simulink model "CLLC"  (R2024a)
settings: Solver=FixedStepAuto  StartTime=0.0  StopTime=0.02  FixedStep=50e-9  RelTol=1e-3
undefined symbols (not defined in the file): DiscIntNeverNeededParam, Ion, Lithium
libraries: spsMosfetLib x8, spsSeriesRLCBranchLib x3, slpidlib x2, simulink x2, spsCurrentMeasurementLib x2, spsBatteryLib x1, spsDCVoltageSourceLib x1, spsLinearTransformerLib x1, spsVoltageMeasurementLib x1, sps_lib x1
settings Model: Creator=DIPAK PRODHANI  LastModifiedBy=DIPAK PRODHANI

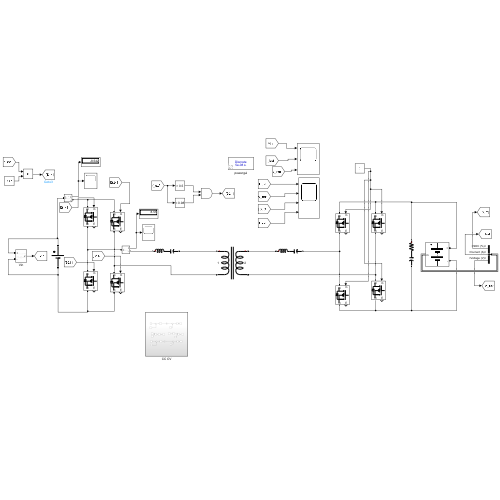
[thumbnail: Simulink's stored preview of the top-level diagram]
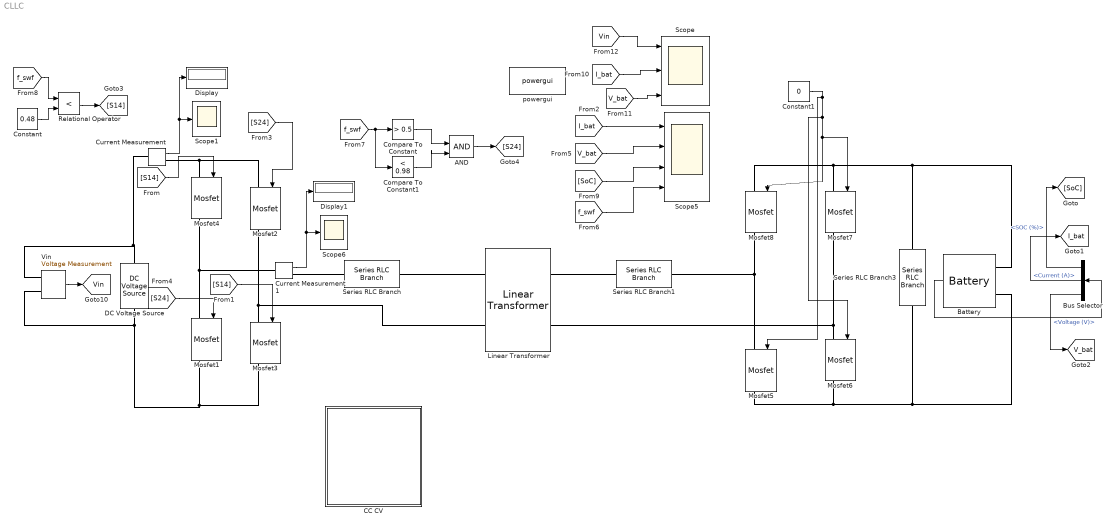
== system CLLC ==
  AND : Logic  IconShape=distinctive  AllPortsSameDT=off  OutDataTypeStr=boolean
  Battery : spsBatteryLib/Battery  BatType=Lithium-Ion  ShowTempParam=off  ThermalPreset=no  ShowAgeParam=off  NomV=720  NomQ=0.0002  SOC=90  Batt_Tr=1e-4  PresetModel=off  MaxQ=0.0002  MinV=540  FullV=838.0707  Dis_rate=8.6957e-05  R=0.5  Normal_OP=0.00018087  expZone="[777.8778  9.826087e-06]"  current=[6.5 13 32.5]  Units=Time  Tci=20  NomT=20  T2=-30  MaxQ2=4.8  FullV2=7.1  Normal_OP2=5.655  expZone2="[6.58           1]"  Rca=0.6  ti=2000  Dp=0  Neq0=0  Tsim=1e6  Ta1=25  Qeol=5.4*0.9  Reol=0.013333*1.2  Char_age=[2.3478, 3]  Dis_age=[2.3478, 10]  N1=1500  N2=10500  N3=1000  N4=1400  Ta2=45  N5=950
  Bus Selector : BusSelector  OutputSignals=SOC (%),Current (A),Voltage (V)
  CC CV : Subsystem
  Compare To Constant : simulink/Logic and Bit Operations/Compare To Constant  relop=>  const=0.5  OutDataTypeStr=boolean
  Compare To Constant1 : simulink/Logic and Bit Operations/Compare To Constant  relop=<  const=0.98  OutDataTypeStr=boolean
  Constant : Constant  Value=0.48
  Constant1 : Constant  Value=0
  Current Measurement : spsCurrentMeasurementLib/Current Measurement  PhasorSimulation=off  OutputType=Complex  PSBequivalent=0
  Current Measurement1 : spsCurrentMeasurementLib/Current Measurement  PhasorSimulation=off  OutputType=Complex  PSBequivalent=0
  DC Voltage Source : spsDCVoltageSourceLib/DC Voltage Source  Amplitude=400  Measurements=None
  Display : Display
  Display1 : Display
  Linear Transformer : spsLinearTransformerLib/Linear Transformer  UNITS=SI  NominalPower=[ 2000 100e3 ]  winding1=[400 0.05 0]  winding2=[615.38 0.1 0]  ThreeWindings=off  winding3=[3.15e+05 0.7938 0.084225]  RmLm=[5000 105.6e-6]  Measurements=None  DataType=on
  Mosfet{1..4} (4 alike) : spsMosfetLib/Mosfet  Ron=0.065  Lon=0  Rd=0.05  Vfd=0.7  IC=0  Rs=1e5  Cs=inf  Measurements=on
  Mosfet{5..8} (4 alike) : spsMosfetLib/Mosfet  Ron=0.08  Lon=0  Rd=0.01  Vfd=0.7  IC=0  Rs=1e5  Cs=inf  Measurements=on
  Relational Operator : RelationalOperator  Operator=<  OutDataTypeStr=boolean  RndMeth=Simplest  InputSameDT=off
  Scope : Scope  NumInputPorts=3
  Scope1 : Scope
  Scope5 : Scope  NumInputPorts=4
  Scope6 : Scope
  Series RLC Branch : spsSeriesRLCBranchLib/Series RLC Branch  LConnTagsString=__new0  RConnTagsString=__new0  BranchType=LC  Resistance=1  Inductance=35.2e-6  SetiL0=off  InitialCurrent=0  Capacitance=71e-9  Setx0=off  InitialVoltage=0  Measurements=None
  Series RLC Branch1 : spsSeriesRLCBranchLib/Series RLC Branch  LConnTagsString=__new0  RConnTagsString=__new0  BranchType=LC  Resistance=1  Inductance=83.31e-6  SetiL0=off  InitialCurrent=0  Capacitance=30e-6  Setx0=off  InitialVoltage=0  Measurements=None
  Series RLC Branch3 : spsSeriesRLCBranchLib/Series RLC Branch  LConnTagsString=__new0  RConnTagsString=__new0  BranchType=RC  Resistance=0.02  Inductance=1e-3  SetiL0=off  InitialCurrent=0  Capacitance=100e-6  Setx0=off  InitialVoltage=0  Measurements=None
  Vin : spsVoltageMeasurementLib/Voltage Measurement  PhasorSimulation=off  OutputType=Complex  PSBequivalent=0
  powergui : sps_lib/powergui  Priority=1  SimulationMode=Discrete  SampleTime=50e-9  frequency=60  Iterations=50  frequencyindice=0  Pbase=100e6  ErrMax=1e-4  UnitsV=kV  UnitsW=MW  buscounter=0  FunctionMessages=off  echomessages=off  EnableUseOfTLC=off  CurrentSourceSwitches=off  DisableSnubberDevices=off  DisableRonSwitches=off  DisableVfSwitches=off  DisplayEquations=off  AutomaticDiscreteSolvers=off  SolverType=Tustin/Backward Euler (TBE)  Interpol=off  ExternalGateDelay=off  methode=off  Ts=100  x0status=blocks  SPID=on  SwTol=0  HookPort=off  NonlinearTolerance=1e-4  nMaxIteration=100  ContinueOnMaxIteration=off  RestoreLinks=warning  ResistiveCurrentMeasurement=off  Frange=[0:2:500]  Ylog=off  Xlog=on  ShowGrid=off  save=off  variable=ZData  structure=0  ZoomFFT=off  StartTime=0.0  cycles=1  DisplayStyle=1  fundamental=60  FreqAxis=off  MaxFrequency=1000  frequencyindicesteady=1  RmsSteady=1  display=off
  tag scope: I_bat=global, V_bat=global, Vin=global
  wires:
  Vin/1 -> [Vin]
  Battery/1 -> Bus Selector/1
  Current Measurement/1 -> Display/1, Scope1/1
  Current Measurement1/1 -> Display1/1, Scope6/1
  Bus Selector/1 -> [SoC]  "<SOC (%)>"
  Bus Selector/2 -> [I_bat]  "<Current (A)>"
  Bus Selector/3 -> [V_bat]  "<Voltage (V)>"
  [f_swf] -> Relational Operator/1
  Constant/1 -> Relational Operator/2
  Relational Operator/1 -> [S14]
  [S14] -> Mosfet4/1
  [S14] -> Mosfet3/1
  [f_swf] -> Compare To Constant1/1, Compare To Constant/1
  Compare To Constant/1 -> AND/1
  Compare To Constant1/1 -> AND/2
  AND/1 -> [S24]
  [S24] -> Mosfet2/1
  [S24] -> Mosfet1/1
  [V_bat] -> Scope/3
  [I_bat] -> Scope/2
  Constant1/1 -> Mosfet5/1, Mosfet6/1, Mosfet7/1, Mosfet8/1
  [I_bat] -> Scope5/1
  [V_bat] -> Scope5/2
  [f_swf] -> Scope5/4
  [SoC] -> Scope5/3
  [Vin] -> Scope/1
  connections:
  Series RLC Branch3/LConn1 -- Battery/LConn1 -- Mosfet7/LConn1 -- Mosfet8/LConn1
  Series RLC Branch3/RConn1 -- Battery/LConn2 -- Mosfet5/RConn1 -- Mosfet6/RConn1
  DC Voltage Source/LConn1 -- Mosfet3/RConn1 -- Mosfet1/RConn1 -- Vin/LConn2
  Linear Transformer/LConn2 -- Mosfet2/RConn1 -- Mosfet3/LConn1
  Linear Transformer/RConn2 -- Mosfet6/LConn1 -- Mosfet7/RConn1
  Vin/LConn1 -- Current Measurement/LConn1 -- DC Voltage Source/RConn1
  Mosfet8/RConn1 -- Series RLC Branch1/RConn1 -- Mosfet5/LConn1
  Mosfet1/LConn1 -- Current Measurement1/LConn1 -- Mosfet4/RConn1
  Series RLC Branch/RConn1 -- Linear Transformer/LConn1
  Series RLC Branch1/LConn1 -- Linear Transformer/RConn1
  Mosfet2/LConn1 -- Current Measurement/RConn1 -- Mosfet4/LConn1
  Current Measurement1/RConn1 -- Series RLC Branch/LConn1

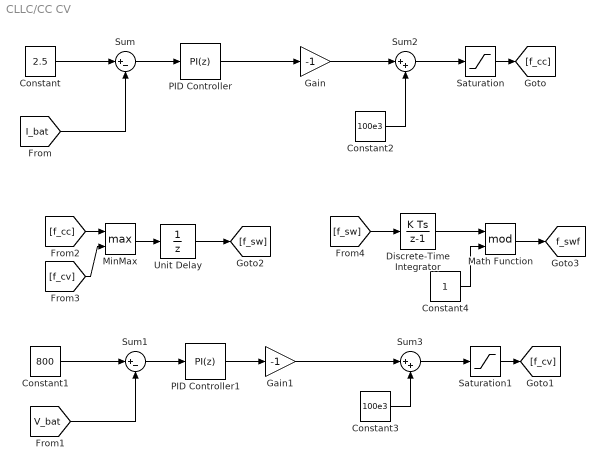
== system CLLC/CC CV ==
  Constant : Constant  Value=2.5
  Constant1 : Constant  Value=800
  Constant2 : Constant  Value=100e3
  Constant3 : Constant  Value=100e3
  Constant4 : Constant
  Discrete-Time Integrator : DiscreteIntegrator  SampleTime=50e-9  ICPrevOutput=DiscIntNeverNeededParam  ICPrevScaledInput=DiscIntNeverNeededParam
  Gain : Gain  Gain=-1
  Gain1 : Gain  Gain=-1
  Math Function : Math  Operator=mod
  MinMax : MinMax  Function=max  Inputs=2
  PID Controller : slpidlib/PID Controller  Controller=PI  Form=Parallel  TimeDomain=Discrete-time  UseExternalTs=off  SampleTime=50e-9  IntegratorMethod=Forward Euler  FilterMethod=Forward Euler  ControllerParametersSource=internal  P=2000  I=500000  UseKiTs=off  D=0  UseExternalDerivativeSource=off  N=100  UseFilter=on  TunerSelectOption=Transfer Function Based (PID Tuner App)  InitialConditionSource=internal  InitialConditionForIntegrator=0  InitialConditionForFilter=0  DifferentiatorICPrevScaledInput=0  ExternalReset=none  TrackingMode=off  Kt=1  LimitOutput=off  SatLimitsSource=internal  UpperSaturationLimit=inf  LowerSaturationLimit=-inf  LinearizeAsGain=on  AntiWindupMode=none  Kb=1  LimitIntegrator=off  UpperIntegratorSaturationLimit=inf  LowerIntegratorSaturationLimit=-inf  POutMin=[]  POutMax=[]  IOutMin=[]  IOutMax=[]  DOutMin=[]  DOutMax=[]  NOutMin=[]  NOutMax=[]  SumOutMin=[]  SumOutMax=[]  SaturationOutMin=[]  SaturationOutMax=[]  PParamMin=[]  PParamMax=[]  IParamMin=[]  IParamMax=[]  DParamMin=[]  DParamMax=[]  NParamMin=[]  NParamMax=[]  KbParamMin=[]  KbParamMax=[]  KtParamMin=[]  KtParamMax=[]  KbOutMin=[]  KbOutMax=[]  KtOutMin=[]  KtOutMax=[]  IntegratorOutMin=[]  IntegratorOutMax=[]  FilterOutMin=[]  FilterOutMax=[]  SumI1OutMin=[]  SumI1OutMax=[]  SumI2OutMin=[]  SumI2OutMax=[]  SumI3OutMin=[]  SumI3OutMax=[]  SumI4OutMin=[]  SumI4OutMax=[]  SumDOutMin=[]  SumDOutMax=[]  DifferentiatorOutMin=[]  DifferentiatorOutMax=[]  FilterDiffOutCoefMin=[]  FilterDiffOutCoefMax=[]  ReciprocalOutMin=[]  ReciprocalOutMax=[]  SumDenOutMin=[]  SumDenOutMax=[]  SumNumOutMin=[]  SumNumOutMax=[]  DivideOutMin=[]  DivideOutMax=[]  UdiffTsProdOutMin=[]  UdiffTsProdOutMax=[]  NTsProdOutMin=[]  NTsProdOutMax=[]  UintegralTsProdOutMin=[]  UintegralTsProdOutMax=[]  UngainTsProdOutMin=[]  UngainTsProdOutMax=[]  ClampingZeroOutDataTypeStr=Inherit: Inherit via back propagation  ClampingZeroOutMin=[]  ClampingZeroOutMax=[]  FilterDenConstantOutDataTypeStr=Inherit: Inherit via back propagation  FilterDenConstantOutMin=[]  FilterDenConstantOutMax=[]  PCopyOutDataTypeStr=Inherit: Inherit via back propagation  PCopyOutMin=[]  PCopyOutMax=[]  NCopyOutDataTypeStr=Inherit: Inherit via back propagation  NCopyOutMin=[]  NCopyOutMax=[]  IntegratorContinuousStateAttributes=''  IntegratorStateMustResolveToSignalObject=off  IntegratorRTWStateStorageClass=Auto  FilterContinuousStateAttributes=''  FilterStateMustResolveToSignalObject=off  FilterRTWStateStorageClass=Auto  ParallelPVariant=InternalParameters  IdealPVariant=Disabled  IVariant=InternalParameters  DVariant=Disabled  IntegratorVariant=Discrete  SatVariant=Disabled  AWVariant=Passthrough  PCopyVariant=Disabled  TRVariant=Disabled  FdbkBlocksVariant=Forward  IdealPFdbkVariant=Disabled  SatFdbkVariant=Disabled  DerivativeFilterVariant=Disabled  NVariant=Disabled  NCopyVariant=Disabled_SignalSpec  FilterICVariant=Disabled  IntegratorICVariant=InternalICs  ExternalResetVariant=Disabled  TRSumVariant=Passthrough  SumFdbkVariant=Disabled  SumVariant=Sum_PI  TsampFilterVariant=InternalTs  TsampNgainVariant=Passthrough  TsampIntegralVariant=Disabled_SignalSpec  ExternalSaturationOutDataTypeStr=Inherit: Same as second input  DerivativeSourceVariant=Disabled
  PID Controller1 : slpidlib/PID Controller  Controller=PI  Form=Parallel  TimeDomain=Discrete-time  UseExternalTs=off  SampleTime=50e-9  IntegratorMethod=Forward Euler  FilterMethod=Forward Euler  ControllerParametersSource=internal  P=200  I=50000  UseKiTs=off  D=0  UseExternalDerivativeSource=off  N=100  UseFilter=on  TunerSelectOption=Transfer Function Based (PID Tuner App)  InitialConditionSource=internal  InitialConditionForIntegrator=0  InitialConditionForFilter=0  DifferentiatorICPrevScaledInput=0  ExternalReset=none  TrackingMode=off  Kt=1  LimitOutput=off  SatLimitsSource=internal  UpperSaturationLimit=inf  LowerSaturationLimit=-inf  LinearizeAsGain=on  AntiWindupMode=none  Kb=1  LimitIntegrator=off  UpperIntegratorSaturationLimit=inf  LowerIntegratorSaturationLimit=-inf  POutMin=[]  POutMax=[]  IOutMin=[]  IOutMax=[]  DOutMin=[]  DOutMax=[]  NOutMin=[]  NOutMax=[]  SumOutMin=[]  SumOutMax=[]  SaturationOutMin=[]  SaturationOutMax=[]  PParamMin=[]  PParamMax=[]  IParamMin=[]  IParamMax=[]  DParamMin=[]  DParamMax=[]  NParamMin=[]  NParamMax=[]  KbParamMin=[]  KbParamMax=[]  KtParamMin=[]  KtParamMax=[]  KbOutMin=[]  KbOutMax=[]  KtOutMin=[]  KtOutMax=[]  IntegratorOutMin=[]  IntegratorOutMax=[]  FilterOutMin=[]  FilterOutMax=[]  SumI1OutMin=[]  SumI1OutMax=[]  SumI2OutMin=[]  SumI2OutMax=[]  SumI3OutMin=[]  SumI3OutMax=[]  SumI4OutMin=[]  SumI4OutMax=[]  SumDOutMin=[]  SumDOutMax=[]  DifferentiatorOutMin=[]  DifferentiatorOutMax=[]  FilterDiffOutCoefMin=[]  FilterDiffOutCoefMax=[]  ReciprocalOutMin=[]  ReciprocalOutMax=[]  SumDenOutMin=[]  SumDenOutMax=[]  SumNumOutMin=[]  SumNumOutMax=[]  DivideOutMin=[]  DivideOutMax=[]  UdiffTsProdOutMin=[]  UdiffTsProdOutMax=[]  NTsProdOutMin=[]  NTsProdOutMax=[]  UintegralTsProdOutMin=[]  UintegralTsProdOutMax=[]  UngainTsProdOutMin=[]  UngainTsProdOutMax=[]  ClampingZeroOutDataTypeStr=Inherit: Inherit via back propagation  ClampingZeroOutMin=[]  ClampingZeroOutMax=[]  FilterDenConstantOutDataTypeStr=Inherit: Inherit via back propagation  FilterDenConstantOutMin=[]  FilterDenConstantOutMax=[]  PCopyOutDataTypeStr=Inherit: Inherit via back propagation  PCopyOutMin=[]  PCopyOutMax=[]  NCopyOutDataTypeStr=Inherit: Inherit via back propagation  NCopyOutMin=[]  NCopyOutMax=[]  IntegratorContinuousStateAttributes=''  IntegratorStateMustResolveToSignalObject=off  IntegratorRTWStateStorageClass=Auto  FilterContinuousStateAttributes=''  FilterStateMustResolveToSignalObject=off  FilterRTWStateStorageClass=Auto  ParallelPVariant=InternalParameters  IdealPVariant=Disabled  IVariant=InternalParameters  DVariant=Disabled  IntegratorVariant=Discrete  SatVariant=Disabled  AWVariant=Passthrough  PCopyVariant=Disabled  TRVariant=Disabled  FdbkBlocksVariant=Forward  IdealPFdbkVariant=Disabled  SatFdbkVariant=Disabled  DerivativeFilterVariant=Disabled  NVariant=Disabled  NCopyVariant=Disabled_SignalSpec  FilterICVariant=Disabled  IntegratorICVariant=InternalICs  ExternalResetVariant=Disabled  TRSumVariant=Passthrough  SumFdbkVariant=Disabled  SumVariant=Sum_PI  TsampFilterVariant=InternalTs  TsampNgainVariant=Passthrough  TsampIntegralVariant=Disabled_SignalSpec  ExternalSaturationOutDataTypeStr=Inherit: Same as second input  DerivativeSourceVariant=Disabled
  Saturation : Saturate  UpperLimit=130e3  LowerLimit=75e3
  Saturation1 : Saturate  UpperLimit=100e3  LowerLimit=75e3
  Sum : Sum  Inputs=|+-
  Sum1 : Sum  Inputs=|+-
  Sum2 : Sum  Inputs=|++
  Sum3 : Sum  Inputs=|++
  Unit Delay : UnitDelay  InitialCondition=100e3  SampleTime=50e-9  HasFrameUpgradeWarning=on
  tag scope: f_swf=global
  wires:
  Constant1/1 -> Sum1/1
  Constant/1 -> Sum/1
  [I_bat] -> Sum/2
  [V_bat] -> Sum1/2
  Sum/1 -> PID Controller/1
  Sum1/1 -> PID Controller1/1
  PID Controller/1 -> Gain/1
  Constant2/1 -> Sum2/2
  Sum2/1 -> Saturation/1
  PID Controller1/1 -> Gain1/1
  Constant3/1 -> Sum3/2
  Sum3/1 -> Saturation1/1
  Gain1/1 -> Sum3/1
  Gain/1 -> Sum2/1
  Saturation1/1 -> [f_cv]
  Saturation/1 -> [f_cc]
  [f_cc] -> MinMax/1
  [f_cv] -> MinMax/2
  MinMax/1 -> Unit Delay/1
  Unit Delay/1 -> [f_sw]
  [f_sw] -> Discrete-Time Integrator/1
  Discrete-Time Integrator/1 -> Math Function/1
  Constant4/1 -> Math Function/2
  Math Function/1 -> [f_swf]
